simulink library "quat_lib"  (R2018b)
settings: Solver=VariableStepAuto  StartTime=0.0  StopTime=10.0  RelTol=1e-3
settings Model: Creator=fabian  LastModifiedBy=yannic

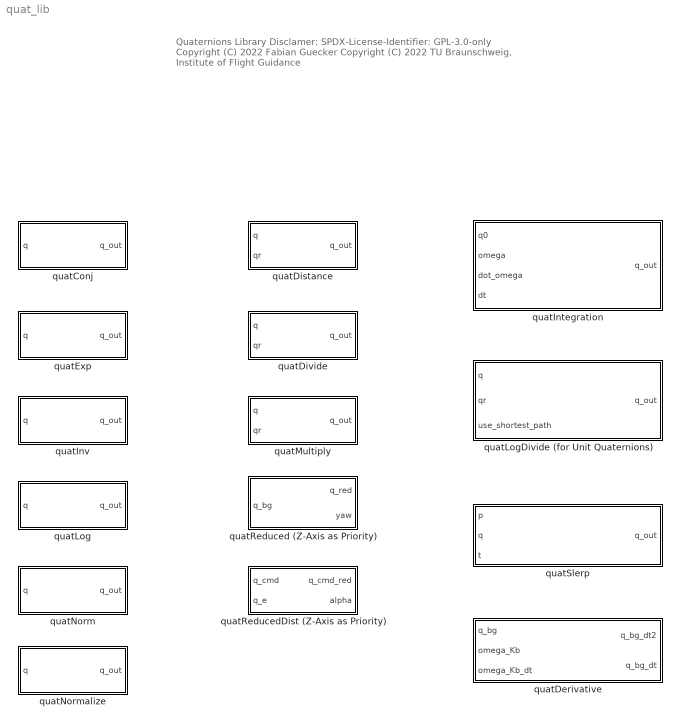
== system quat_lib ==
  note: Quaternions Library
      |
      | Disclamer:
      | SPDX-License-Identifier: GPL-3.0-only
      |
      | Copyright (C) 2022 Fabian Guecker
      | Copyright (C) 2022 TU Braunschweig, Institute of Flight Guidance
  quatConj : MATLAB Function  TreatAsAtomicUnit=on
  quatDerivative : MATLAB Function  TreatAsAtomicUnit=on
  quatDistance : MATLAB Function  TreatAsAtomicUnit=on
  quatDivide : MATLAB Function  TreatAsAtomicUnit=on
  quatExp : MATLAB Function  TreatAsAtomicUnit=on
  quatIntegration : MATLAB Function  TreatAsAtomicUnit=on
  quatInv : MATLAB Function  TreatAsAtomicUnit=on
  quatLog : MATLAB Function  TreatAsAtomicUnit=on
  quatLogDivide (for Unit Quaternions) : MATLAB Function  TreatAsAtomicUnit=on
  quatMultiply : MATLAB Function  TreatAsAtomicUnit=on
  quatNorm : MATLAB Function  TreatAsAtomicUnit=on
  quatNormalize : MATLAB Function  TreatAsAtomicUnit=on
  quatReduced (Z-Axis as Priority) : MATLAB Function  TreatAsAtomicUnit=on
  quatReducedDist (Z-Axis as Priority) : MATLAB Function  TreatAsAtomicUnit=on
  quatSlerp : MATLAB Function  TreatAsAtomicUnit=on

== matlab function quat_lib/quatDistance ==
  data: q input size=4; q_out output; qr input size=4
function q_out = quatDistance(q, qr)

q_out = quatDistance(q, qr);

end

== matlab function quat_lib/quatConj ==
  data: q input size=4; q_out output
function q_out = quatConj( q )

q_out = quatConj( q );

end

== matlab function quat_lib/quatDivide ==
  data: q input size=4; q_out output; qr input size=4
function q_out = quatDivide(q, qr)

q_out = quatDivide(q, qr);

end

== matlab function quat_lib/quatExp ==
  data: q input size=4; q_out output
function q_out = quatExp( q )

q_out = quatExp( q );

end

== matlab function quat_lib/quatLog ==
  data: q input size=4; q_out output
function q_out = quatLog( q )

q_out = quatLog( q );

end

== matlab function quat_lib/quatInv ==
  data: q input size=4; q_out output
function q_out = quatInv( q )

q_out = quatInv( q );

end

== matlab function quat_lib/quatNorm ==
  data: q input size=4; q_out output
function q_out = quatNorm( q )

q_out = quatNorm( q );

end

== matlab function quat_lib/quatNormalize ==
  data: q input size=4; q_out output
function q_out = quatNormalize( q )

q_out = quatNormalize( q );

end

== matlab function quat_lib/quatMultiply ==
  data: q input size=4; q_out output; qr input size=4
function q_out = quatMultiply(q, qr)

q_out = quatMultiply(q, qr);

end

== matlab function quat_lib/quatReducedDist (Z-Axis as Priority) ==
  data: q_cmd input size=4; q_cmd_red output; q_e input size=4; alpha output
function [q_cmd_red, alpha] = quatReducedDist(q_cmd, q_e)

[q_cmd_red, alpha] = quatReducedDist(q_cmd, q_e);

end

== matlab function quat_lib/quatIntegration ==
  data: q0 input size=4; q_out output; omega input size=3; dot_omega input size=3; dt input size=1
function q_out = quatIntegration(q0, omega, dot_omega, dt)

q_out = quatIntegration(q0, omega, dot_omega, dt);

end

== matlab function quat_lib/quatLogDivide (for Unit Quaternions) ==
  data: q input size=4; q_out output; qr input size=4; use_shortest_path input size=1
function q_out = quatLogDivide(q, qr, use_shortest_path)

q_out = quatLogDivide(q, qr, use_shortest_path);

end

== matlab function quat_lib/quatReduced (Z-Axis as Priority) ==
  data: q_bg input size=4; q_red output; yaw output
function [q_red,yaw] = quatReduced(q_bg)

[q_red,yaw] = quatReduced(q_bg);

end

== matlab function quat_lib/quatSlerp ==
  data: p input size=4; q_out output; q input size=4; t input size=1
function q_out  = quatSlerp(p, q, t)

[q_out] = quatSlerp(p, q, t);

end

== matlab function quat_lib/quatDerivative ==
  data: q_bg input size=4; q_bg_dt2 output; q_bg_dt output; omega_Kb input; omega_Kb_dt input
function [q_bg_dt2,q_bg_dt] = quatDerivative( q_bg, omega_Kb, omega_Kb_dt )

[q_bg_dt2,q_bg_dt] = quatDerivative( q_bg, omega_Kb, omega_Kb_dt );

end
